simulink model "Lcc"  (R2022b)
settings: Solver=ode45  StartTime=0.0  StopTime=10.0  RelTol=1e-3  EnableMultiTasking=on
undefined symbols (not defined in the file): Lcc_facInitValue, Lcc_flgLambdaControlActive, Lcc_flgSwitch2PIDController, Lcc_IntStartValueTPC, Lcc_LambdaCorrMaxPID, Lcc_LambdaCorrMaxTPC, Lcc_LambdaCorrMinPID, Lcc_LambdaCorrMinTPC, Lcc_StartValuePID
libraries: simulink x6
settings Model: Creator=YAL9FE  LastModifiedBy=ZJO9FE
settings SolverCC: AlgebraicLoopSolver=TrustRegion
settings DataIOCC: LimitDataPoints=on  SaveFormat=Array  SignalLoggingSaveFormat=ModelDataLogs  ReturnWorkspaceOutputs=off
settings OptimizationCC: ExpressionDepthLimit=2147483647  LifeSpan=inf
settings DebuggingCC: UnderspecifiedInitializationDetection=Classic  MergeDetectMultiDrivingBlocksExec=none  SolverPrmCheckMsg=warning  FcnCallInpInsideContextMsg=warning  UnconnectedInputMsg=warning  UnconnectedOutputMsg=warning  UnconnectedLineMsg=warning  StateNameClashWarn=warning  SFUnexpectedBacktrackingDiag=warning  SFNoUnconditionalDefaultTransitionDiag=warning  SFExecutionAtInitializationDiag=none  SFMachineParentedDataDiag=warning  ArithmeticOperatorsInVariantConditions=warning
settings HardwareCC: ProdBitPerPointer=32  ProdBitPerSizeT=32  ProdBitPerPtrDiffT=32  ProdLargestAtomicFloat=None  ProdIntDivRoundTo=Undefined  ProdEndianess=Unspecified  ProdWordSize=32  ProdHWDeviceType=32-bit Generic
settings ModelReferenceCC: EnableRefExpFcnMdlSchedulingChecks=on  PropagateSignalLabelsOutOfModel=off
settings SFSimCC: SimUseLocalCustomCode=off  CustomCodeUndefinedFunction=UseInterfaceOnly
settings RTWCC: RTWUseLocalCustomCode=off
settings CodeAppCC: StateflowObjectComments=on
settings GRTTargetCC: TargetLangStandard=C89/C90 (ANSI)  CombineOutputUpdateFcns=off  GRTInterface=on
settings ConfigComp: CovMetricSettings=dw  CovSaveCumulativeToWorkspaceVar=on  CovSaveSingleToWorkspaceVar=on  CovExternalEMLEnable=off  CovSFcnEnable=off

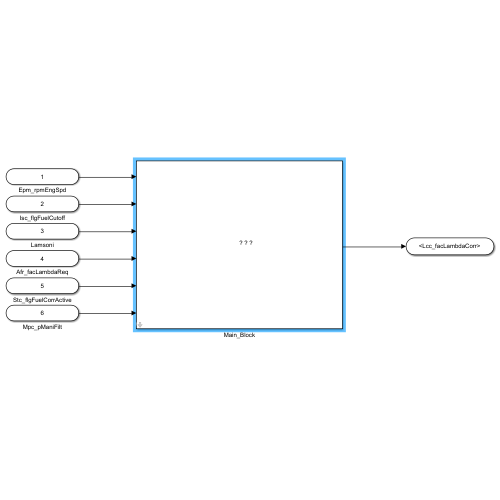
[thumbnail: Simulink's stored preview of the top-level diagram]
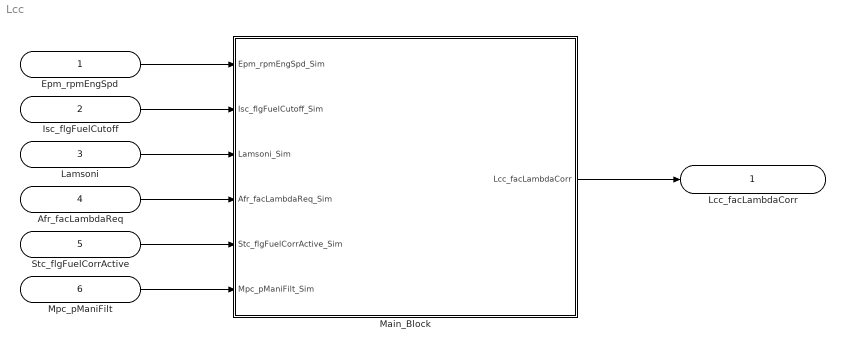
== system Lcc ==
  Epm_rpmEngSpd : Inport
  Isc_flgFuelCutoff : Inport  Port=2
  Lamsoni : Inport  Port=3
  Afr_facLambdaReq : Inport  Port=4
  Stc_flgFuelCorrActive : Inport  Port=5
  Mpc_pManiFilt : Inport  Port=6
  Main_Block : Subsystem  mask(Functions){}
      mask help: LambdaControl
      mask Display:
      | image(imread('LambdaControl.jpg'))
      | port_label('input',1,'Epm_rpmEngSpd_Sim')
      | port_label('input',2,'Isc_flgFuelCutoff_Sim')
      | port_label('input',3,'Lamsoni_Sim')
      | port_label('input',4,'Afr_facLambdaReq_Sim')
      | port_label('input',5,'Stc_flgFuelCorrActive_Sim')
      | port_label('input',6,'Mpc_pManiFilt_Sim')
      | port_label('output',1,'Lcc_facLambdaCorr_Sim')
  Lcc_facLambdaCorr : Outport
  wires:
  Main_Block/1(Lcc_facLambdaCorr) -> Lcc_facLambdaCorr/1
  Epm_rpmEngSpd/1 -> Main_Block/1(Epm_rpmEngSpd_Sim)
  Isc_flgFuelCutoff/1 -> Main_Block/2(Isc_flgFuelCutoff_Sim)
  Lamsoni/1 -> Main_Block/3(Lamsoni_Sim)
  Afr_facLambdaReq/1 -> Main_Block/4(Afr_facLambdaReq_Sim)
  Stc_flgFuelCorrActive/1 -> Main_Block/5(Stc_flgFuelCorrActive_Sim)
  Mpc_pManiFilt/1 -> Main_Block/6(Mpc_pManiFilt_Sim)

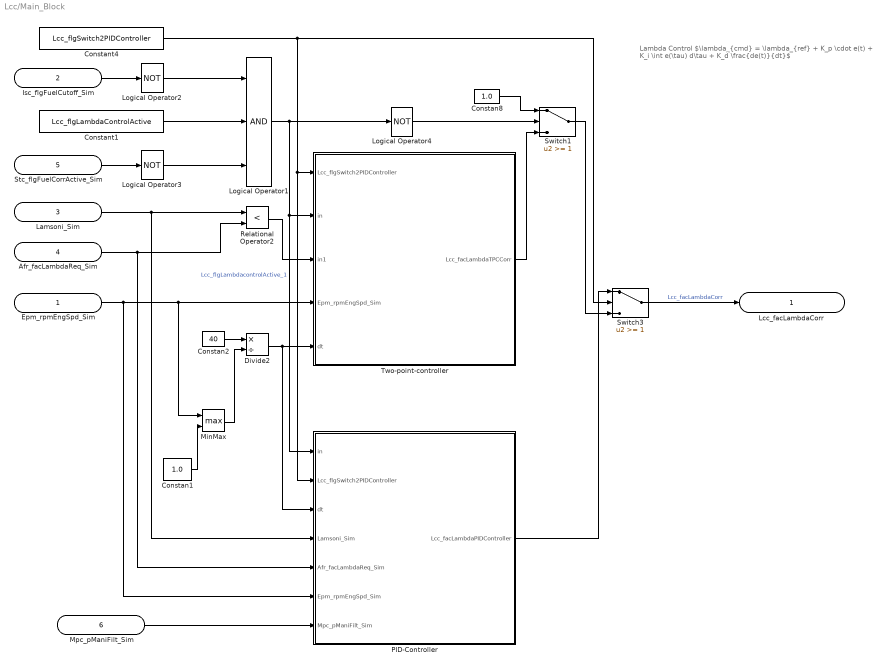
== system Lcc/Main_Block ==
  note: Lambda Control
      | $\lambda_{cmd} = \lambda_{ref} + K_p \cdot e(t) + K_i \int e(\tau) d\tau + K_d \frac{de(t)}{dt}$
  Epm_rpmEngSpd_Sim : Inport
  Isc_flgFuelCutoff_Sim : Inport  Port=2
  Lamsoni_Sim : Inport  Port=3
  Afr_facLambdaReq_Sim : Inport  Port=4
  Stc_flgFuelCorrActive_Sim : Inport  Port=5
  Mpc_pManiFilt_Sim : Inport  Port=6
  Constan1 : Constant  Value=1.0  OutDataTypeStr=single
  Constan2 : Constant  Value=40  OutDataTypeStr=single
  Constan8 : Constant  Value=1.0  OutDataTypeStr=single
  Constant1 : Constant  Value=Lcc_flgLambdaControlActive
  Constant4 : Constant  Value=Lcc_flgSwitch2PIDController
  Divide2 : Product  Inputs=*/  OutDataTypeStr=Inherit: Same as first input
  Logical Operator1 : Logic  Inputs=3  AllPortsSameDT=off  OutDataTypeStr=boolean
  Logical Operator2 : Logic  Operator=NOT  AllPortsSameDT=off  OutDataTypeStr=boolean
  Logical Operator3 : Logic  Operator=NOT  AllPortsSameDT=off  OutDataTypeStr=boolean
  Logical Operator4 : Logic  Operator=NOT  AllPortsSameDT=off  OutDataTypeStr=boolean
  MinMax : MinMax  Function=max  Inputs=2
  PID-Controller : Subsystem
  Relational Operator2 : RelationalOperator  Operator=<  OutDataTypeStr=boolean  InputSameDT=off
  Switch1 : Switch  Threshold=1  SaturateOnIntegerOverflow=off  InputSameDT=off
  Switch3 : Switch  Threshold=1  SaturateOnIntegerOverflow=off  InputSameDT=off
  Two-point-controller : Subsystem
  Lcc_facLambdaCorr : Outport
  wires:
  Isc_flgFuelCutoff_Sim/1 -> Logical Operator2/1
  Stc_flgFuelCorrActive_Sim/1 -> Logical Operator3/1
  Logical Operator2/1 -> Logical Operator1/1
  Logical Operator3/1 -> Logical Operator1/3
  Constant1/1 -> Logical Operator1/2
  Logical Operator1/1 -> Logical Operator4/1, Two-point-controller/2(in), PID-Controller/1(in)  "Lcc_flgLambdacontrolActive_1"
  Logical Operator4/1 -> Switch1/2
  Constan8/1 -> Switch1/1
  Constant4/1 -> Switch3/2, Two-point-controller/1(Lcc_flgSwitch2PIDController), PID-Controller/2(Lcc_flgSwitch2PIDController)
  Switch1/1 -> Switch3/3
  Switch3/1 -> Lcc_facLambdaCorr/1  "Lcc_facLambdaCorr"
  Lamsoni_Sim/1 -> Relational Operator2/1, PID-Controller/4(Lamsoni_Sim)
  Afr_facLambdaReq_Sim/1 -> Relational Operator2/2, PID-Controller/5(Afr_facLambdaReq_Sim)
  Epm_rpmEngSpd_Sim/1 -> MinMax/1, Two-point-controller/4(Epm_rpmEngSpd_Sim), PID-Controller/6(Epm_rpmEngSpd_Sim)
  Constan2/1 -> Divide2/1
  Constan1/1 -> MinMax/2
  MinMax/1 -> Divide2/2
  Two-point-controller/1(Lcc_facLambdaTPCCorr) -> Switch1/3
  Relational Operator2/1 -> Two-point-controller/3(in1)
  Divide2/1 -> Two-point-controller/5(dt), PID-Controller/3(dt)
  PID-Controller/1(Lcc_facLambdaPIDController) -> Switch3/1
  Mpc_pManiFilt_Sim/1 -> PID-Controller/7(Mpc_pManiFilt_Sim)

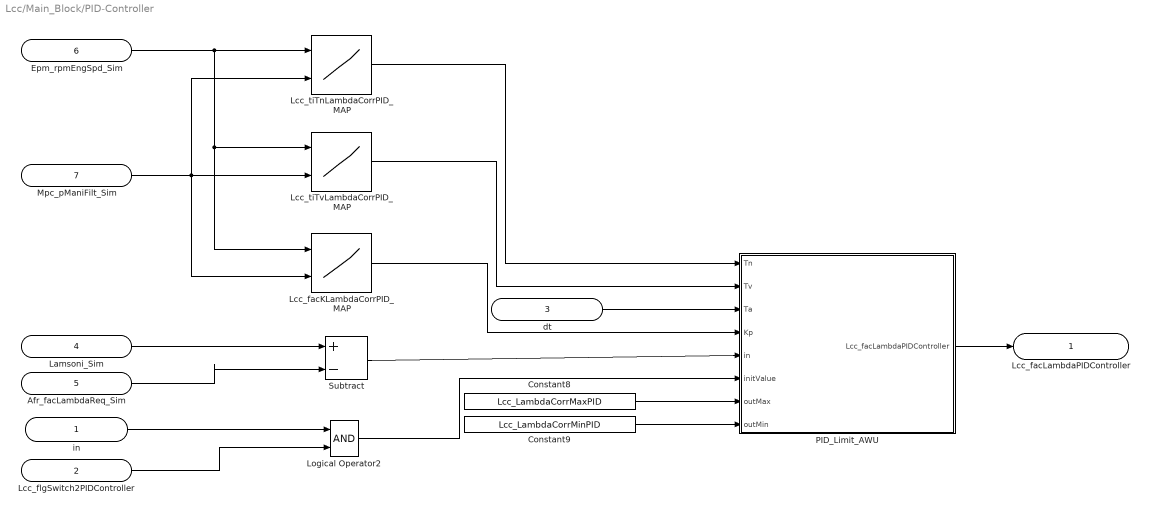
== system Lcc/Main_Block/PID-Controller ==
  in : Inport
  Lcc_flgSwitch2PIDController : Inport  Port=2
  dt : Inport  Port=3
  Lamsoni_Sim : Inport  Port=4
  Afr_facLambdaReq_Sim : Inport  Port=5
  Epm_rpmEngSpd_Sim : Inport  Port=6
  Mpc_pManiFilt_Sim : Inport  Port=7
  Constant8 : Constant  Value=Lcc_LambdaCorrMaxPID
  Constant9 : Constant  Value=Lcc_LambdaCorrMinPID
  Lcc_facKLambdaCorrPID_MAP : Lookup_n-D  BreakpointsForDimension1=[1:3]  BreakpointsForDimension2=[1:3]  Table=[1 3 5;3 6 8;1 2 3]  ExtrapMethod=Clip
      settings: InputPortMap=u0,u1
  Lcc_tiTnLambdaCorrPID_MAP : Lookup_n-D  BreakpointsForDimension1=[1:3]  BreakpointsForDimension2=[1:3]  Table=[1 3 5;3 6 8;1 2 3]  ExtrapMethod=Clip
      settings: InputPortMap=u0,u1
  Lcc_tiTvLambdaCorrPID_MAP : Lookup_n-D  BreakpointsForDimension1=[1:3]  BreakpointsForDimension2=[1:3]  Table=[1 3 5;3 6 8;1 2 3]  ExtrapMethod=Clip
      settings: InputPortMap=u0,u1
  Logical Operator2 : Logic  AllPortsSameDT=off  OutDataTypeStr=boolean
  PID_Limit_AWU : Subsystem
      mask help: PID_Limit_AWU
      mask Display: image(imread('PID_Limit_AWU.jpg'))
  Subtract : Sum  Inputs=+-  OutDataTypeStr=Inherit: Same as first input
  Lcc_facLambdaPIDController : Outport
  wires:
  PID_Limit_AWU/1(Lcc_facLambdaPIDController) -> Lcc_facLambdaPIDController/1
  Epm_rpmEngSpd_Sim/1 -> Lcc_tiTnLambdaCorrPID_MAP/1, Lcc_tiTvLambdaCorrPID_MAP/1, Lcc_facKLambdaCorrPID_MAP/1
  Mpc_pManiFilt_Sim/1 -> Lcc_tiTnLambdaCorrPID_MAP/2, Lcc_tiTvLambdaCorrPID_MAP/2, Lcc_facKLambdaCorrPID_MAP/2
  Lcc_tiTnLambdaCorrPID_MAP/1 -> PID_Limit_AWU/1(Tn)
  Lcc_tiTvLambdaCorrPID_MAP/1 -> PID_Limit_AWU/2(Tv)
  dt/1 -> PID_Limit_AWU/3(Ta)
  Lcc_facKLambdaCorrPID_MAP/1 -> PID_Limit_AWU/4(Kp)
  Subtract/1 -> PID_Limit_AWU/5(in)
  Constant8/1 -> PID_Limit_AWU/7(outMax)
  Constant9/1 -> PID_Limit_AWU/8(outMin)
  Lamsoni_Sim/1 -> Subtract/1
  Afr_facLambdaReq_Sim/1 -> Subtract/2
  in/1 -> Logical Operator2/1
  Lcc_flgSwitch2PIDController/1 -> Logical Operator2/2
  Logical Operator2/1 -> PID_Limit_AWU/6(initValue)

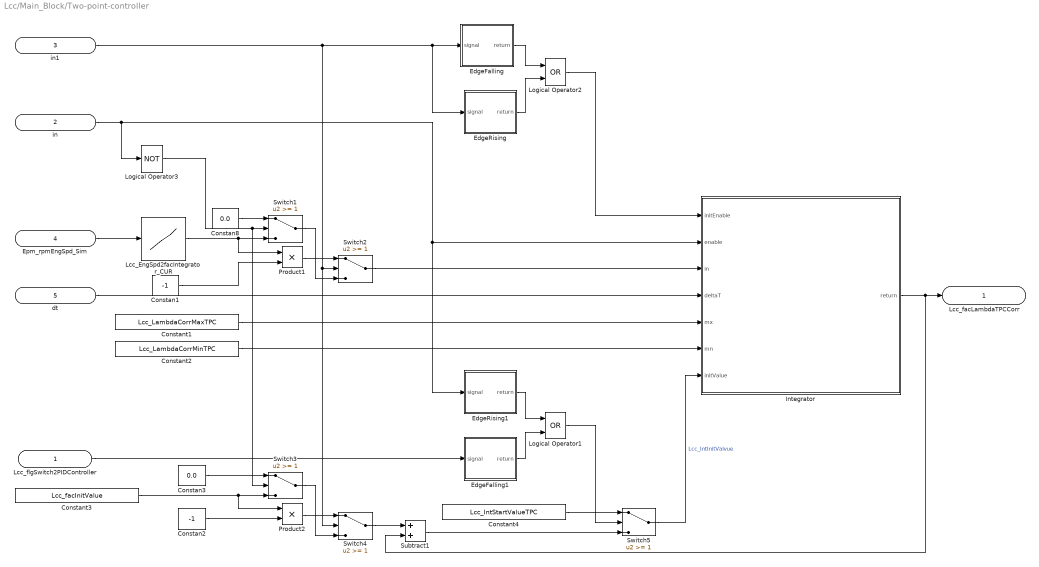
== system Lcc/Main_Block/Two-point-controller ==
  Lcc_flgSwitch2PIDController : Inport
  in : Inport  Port=2
  in1 : Inport  Port=3
  Epm_rpmEngSpd_Sim : Inport  Port=4
  dt : Inport  Port=5
  Constan1 : Constant  Value=-1  OutDataTypeStr=single
  Constan2 : Constant  Value=-1  OutDataTypeStr=single
  Constan3 : Constant  Value=0.0  OutDataTypeStr=single
  Constan8 : Constant  Value=0.0  OutDataTypeStr=single
  Constant1 : Constant  Value=Lcc_LambdaCorrMaxTPC
  Constant2 : Constant  Value=Lcc_LambdaCorrMinTPC
  Constant3 : Constant  Value=Lcc_facInitValue
  Constant4 : Constant  Value=Lcc_IntStartValueTPC
  EdgeFalling : Subsystem
      mask help: EdgeFalling
      mask Display: image(imread('EdgeFalling.jpg'))
  EdgeFalling1 : Subsystem
      mask help: EdgeFalling
      mask Display: image(imread('EdgeFalling.jpg'))
  EdgeRising : Subsystem
      mask help: EdgeRising
      mask Display: image(imread('EdgeRising.jpg'))
  EdgeRising1 : Subsystem
      mask help: EdgeRising
      mask Display: image(imread('EdgeRising.jpg'))
  Integrator : Subsystem
      mask help: Integrator
      mask Display: image(imread('Integrator.jpg'))
  Lcc_EngSpd2facIntegrator_CUR : Lookup_n-D  NumberOfTableDimensions=1  BreakpointsForDimension1=[1:3]  Table=[4 5 8]  ExtrapMethod=Clip
  Logical Operator1 : Logic  Operator=OR  AllPortsSameDT=off  OutDataTypeStr=boolean
  Logical Operator2 : Logic  Operator=OR  AllPortsSameDT=off  OutDataTypeStr=boolean
  Logical Operator3 : Logic  Operator=NOT  AllPortsSameDT=off  OutDataTypeStr=boolean
  Product1 : Product  OutDataTypeStr=Inherit: Same as first input
  Product2 : Product  OutDataTypeStr=Inherit: Same as first input
  Subtract1 : Sum  OutDataTypeStr=Inherit: Same as first input
  Switch{1..5} (5 alike) : Switch  Threshold=1  SaturateOnIntegerOverflow=off  InputSameDT=off
  Lcc_facLambdaTPCCorr : Outport
  wires:
  EdgeFalling/1(return) -> Logical Operator2/1
  EdgeRising/1(return) -> Logical Operator2/2
  in1/1 -> EdgeFalling/1(signal), EdgeRising/1(signal), Switch2/2, Switch4/2
  EdgeRising1/1(return) -> Logical Operator1/1
  EdgeFalling1/1(return) -> Logical Operator1/2
  in/1 -> Logical Operator3/1, Integrator/2(enable), EdgeRising1/1(signal)
  Logical Operator3/1 -> Switch1/2, Switch3/2
  Epm_rpmEngSpd_Sim/1 -> Lcc_EngSpd2facIntegrator_CUR/1
  Lcc_EngSpd2facIntegrator_CUR/1 -> Switch1/3, Product1/1
  Constan8/1 -> Switch1/1
  Switch1/1 -> Switch2/3
  Product1/1 -> Switch2/1
  Constan1/1 -> Product1/2
  Constant3/1 -> Product2/1, Switch3/3
  Switch3/1 -> Switch4/3
  Product2/1 -> Switch4/1
  Constan2/1 -> Product2/2
  Constan3/1 -> Switch3/1
  Switch4/1 -> Subtract1/1
  Logical Operator1/1 -> Switch5/2
  Subtract1/1 -> Switch5/3
  Constant4/1 -> Switch5/1
  Integrator/1(return) -> Lcc_facLambdaTPCCorr/1, Subtract1/2
  Logical Operator2/1 -> Integrator/1(initEnable)
  Switch2/1 -> Integrator/3(in)
  dt/1 -> Integrator/4(deltaT)
  Switch5/1 -> Integrator/7(initValue)  "Lcc_IntInitValvue"
  Constant1/1 -> Integrator/5(mx)
  Constant2/1 -> Integrator/6(mn)
  Lcc_flgSwitch2PIDController/1 -> EdgeFalling1/1(signal)

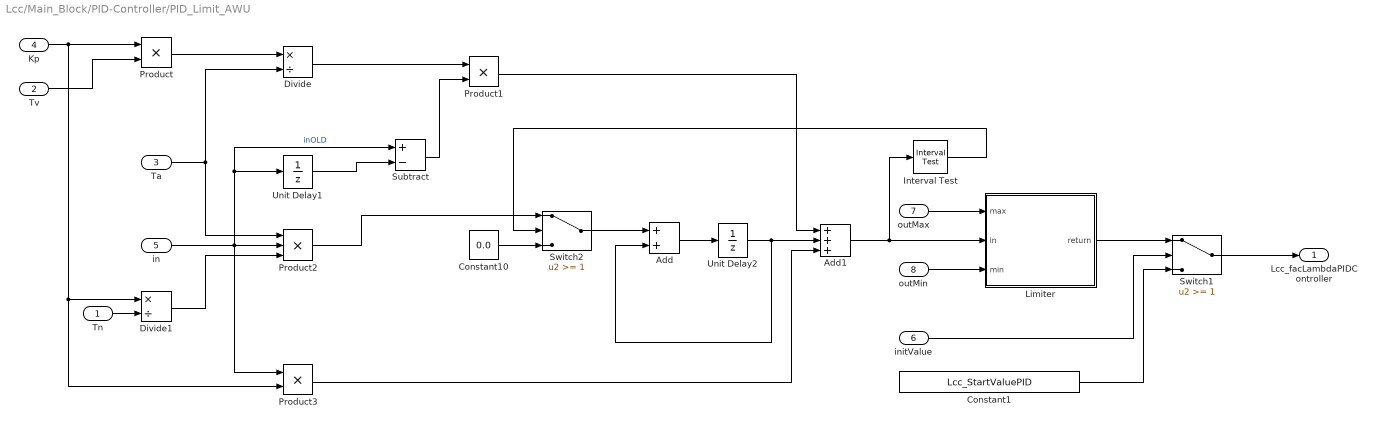
== system Lcc/Main_Block/PID-Controller/PID_Limit_AWU ==
  Tn : Inport
  Tv : Inport  Port=2
  Ta : Inport  Port=3
  Kp : Inport  Port=4
  in : Inport  Port=5
  initValue : Inport  Port=6
  outMax : Inport  Port=7
  outMin : Inport  Port=8
  Add : Sum  OutDataTypeStr=Inherit: Same as first input
  Add1 : Sum  Inputs=+++  OutDataTypeStr=Inherit: Same as first input
  Constant1 : Constant  Value=Lcc_StartValuePID
  Constant10 : Constant  Value=0.0  OutDataTypeStr=single
  Divide : Product  Inputs=*/  OutDataTypeStr=Inherit: Same as first input
  Divide1 : Product  Inputs=*/  OutDataTypeStr=Inherit: Same as first input
  Interval Test : simulink/Logic and Bit Operations/Interval Test  IntervalClosedRight=on  uplimit=Lcc_LambdaCorrMaxPID  IntervalClosedLeft=on  lowlimit=Lcc_LambdaCorrMinPID  OutDataTypeStr=boolean
  Limiter : Subsystem
      mask help: Limiter
      mask Display: image(imread('Limiter.jpg'))
  Product : Product  OutDataTypeStr=Inherit: Same as first input
  Product1 : Product  OutDataTypeStr=Inherit: Same as first input
  Product2 : Product  Inputs=3  OutDataTypeStr=Inherit: Same as first input
  Product3 : Product  OutDataTypeStr=Inherit: Same as first input
  Subtract : Sum  Inputs=+-  OutDataTypeStr=Inherit: Same as first input
  Switch1 : Switch  Threshold=1  SaturateOnIntegerOverflow=off  InputSameDT=off
  Switch2 : Switch  Threshold=1  SaturateOnIntegerOverflow=off  InputSameDT=off
  Unit Delay1 : UnitDelay  SampleTime=-1  HasFrameUpgradeWarning=on
  Unit Delay2 : UnitDelay  SampleTime=-1  HasFrameUpgradeWarning=on
  Lcc_facLambdaPIDController : Outport
  wires:
  Constant10/1 -> Switch2/3
  Product2/1 -> Switch2/1
  Interval Test/1 -> Switch2/2
  Unit Delay2/1 -> Add/2, Add1/2
  Add/1 -> Unit Delay2/1
  Unit Delay1/1 -> Subtract/2
  Kp/1 -> Product/1, Product3/2, Divide1/1
  Tv/1 -> Product/2
  Product/1 -> Divide/1
  Ta/1 -> Product2/1, Divide/2
  Divide/1 -> Product1/1
  Tn/1 -> Divide1/2
  in/1 -> Product2/2, Product3/1, Subtract/1, Unit Delay1/1  "inOLD"
  Divide1/1 -> Product2/3
  Subtract/1 -> Product1/2
  Switch2/1 -> Add/1
  Product3/1 -> Add1/3
  Product1/1 -> Add1/1
  Add1/1 -> Limiter/2(in), Interval Test/1
  outMin/1 -> Limiter/3(min)
  outMax/1 -> Limiter/1(max)
  Switch1/1 -> Lcc_facLambdaPIDController/1
  initValue/1 -> Switch1/2
  Limiter/1(return) -> Switch1/1
  Constant1/1 -> Switch1/3

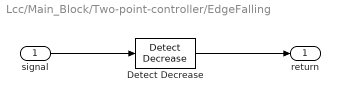
== system Lcc/Main_Block/Two-point-controller/EdgeFalling ==
  signal : Inport
  Detect Decrease : simulink/Logic and Bit Operations/Detect Decrease  vinit=0.0  InputProcessing=Inherited  OutDataTypeStr=boolean
  return : Outport
  wires:
  Detect Decrease/1 -> return/1
  signal/1 -> Detect Decrease/1

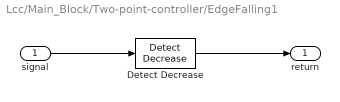
== system Lcc/Main_Block/Two-point-controller/EdgeFalling1 ==
  signal : Inport
  Detect Decrease : simulink/Logic and Bit Operations/Detect Decrease  vinit=0.0  InputProcessing=Inherited  OutDataTypeStr=boolean
  return : Outport
  wires:
  signal/1 -> Detect Decrease/1
  Detect Decrease/1 -> return/1

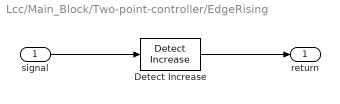
== system Lcc/Main_Block/Two-point-controller/EdgeRising ==
  signal : Inport
  Detect Increase : simulink/Logic and Bit Operations/Detect Increase  vinit=0.0  InputProcessing=Inherited  OutDataTypeStr=boolean
  return : Outport
  wires:
  Detect Increase/1 -> return/1
  signal/1 -> Detect Increase/1

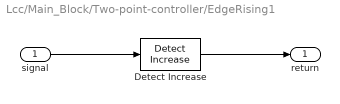
== system Lcc/Main_Block/Two-point-controller/EdgeRising1 ==
  signal : Inport
  Detect Increase : simulink/Logic and Bit Operations/Detect Increase  vinit=0.0  InputProcessing=Inherited  OutDataTypeStr=boolean
  return : Outport
  wires:
  signal/1 -> Detect Increase/1
  Detect Increase/1 -> return/1

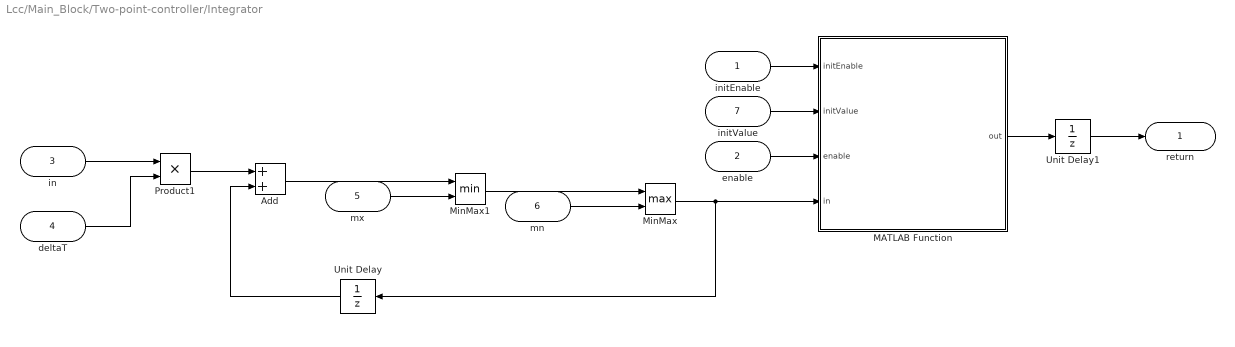
== system Lcc/Main_Block/Two-point-controller/Integrator ==
  initEnable : Inport
  enable : Inport  Port=2
  in : Inport  Port=3
  deltaT : Inport  Port=4
  mx : Inport  Port=5
  mn : Inport  Port=6
  initValue : Inport  Port=7
  Add : Sum
  MATLAB Function : MATLAB Function  TreatAsAtomicUnit=on
  MinMax : MinMax  Function=max  Inputs=2
  MinMax1 : MinMax  Inputs=2
  Product1 : Product  OutDataTypeStr=Inherit: Same as first input
  Unit Delay : UnitDelay  SampleTime=-1  HasFrameUpgradeWarning=on
  Unit Delay1 : UnitDelay  SampleTime=-1  HasFrameUpgradeWarning=on
  return : Outport
  wires:
  deltaT/1 -> Product1/2
  in/1 -> Product1/1
  Product1/1 -> Add/1
  Add/1 -> MinMax1/1
  mx/1 -> MinMax1/2
  MinMax1/1 -> MinMax/1
  mn/1 -> MinMax/2
  Unit Delay/1 -> Add/2
  MinMax/1 -> Unit Delay/1, MATLAB Function/4(in)
  MATLAB Function/1(out) -> Unit Delay1/1
  enable/1 -> MATLAB Function/3(enable)
  initValue/1 -> MATLAB Function/2(initValue)
  initEnable/1 -> MATLAB Function/1(initEnable)
  Unit Delay1/1 -> return/1

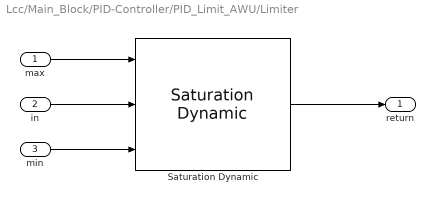
== system Lcc/Main_Block/PID-Controller/PID_Limit_AWU/Limiter ==
  max : Inport
  in : Inport  Port=2
  min : Inport  Port=3
  Saturation Dynamic : simulink/Discontinuities/Saturation Dynamic  OutMin=[]  OutMax=[]  OutDataTypeStr=Inherit: Same as second input  OutDataType=fixdt(1, 16)  OutScaling=2^-10  DoSatur=off
  return : Outport
  wires:
  max/1 -> Saturation Dynamic/1
  in/1 -> Saturation Dynamic/2
  min/1 -> Saturation Dynamic/3
  Saturation Dynamic/1 -> return/1

== matlab function Lcc/Main_Block/Two-point-controller/Integrator/MATLAB Function ==
  data: initEnable input; out output; initValue input; enable input; in input
function out = fcn(initEnable,initValue,enable,in)
% Integrator Test
out = single(0.0);
if(initEnable==true)
    out = initValue;
end
if(enable==true)
    out = single(in);
end
